simulink model "hrg_lift_tdm_shared"  (R2025a)
settings: Solver=FixedStepDiscrete  StartTime=0.0  StopTime=(floor(c.duration/L.T+1e-9)-1)*L.T  FixedStep=L.T  RelTol=1e-3
model workspace (MAT data in the model file):
  L.F = [0.999580432532 -1.0372095128e-09 6.81624270452e-05 6.2277917735e-05 1.75963318556e-117 1.36918786801e-121 -0.235732623336 -0.000170581053866 0.235732623336 0.000170581053866 8.59950268771e-05 -1.70759216614e-09 ... (676 elements, 26x26)]
  L.G = [-0.000674269741511 -4.08813584994e-07 0.00751103389356 -4.57676319434e-08 1.57194245886e-96 -1.68771046318e-124 -0.0205539124342 2.21019907253e-07 0.0205539124342 -2.21019907253e-07 -3.00124965015e-07 -2.89912617394e-11 ... (104 elements, 26x4)]
  L.Hm = [0.999684195246  -1.23947288142e-06  -4.2771939927e-05  -4.66937085047e-05  -1.75385746799e-05  -9.52623491396e-09  -2.77437214297e-15  -3.69811119948e-16  2.77437214289e-15  3.69811119948e-16  0  0  0  0  0  0  0  0  0  0  0  0  0  0  0  0; -1.23947288142e-06  0.999686910144  -4.66937085048e-05  5.9504357854e-05  -9.52623491397e-09  -1.75177087416e-05  -3.69811119948e-16  -1.96435054823e-15  3.69811119948e-16  1.96435054816e-15  0  0  0  0  0  0  0  0  0  0  0  0  0  0  0  0; 7.61670764012e-05  4.67132902328e-05  0.999689500075  3.71691546591e-06  0.000204402550454  -5.17736492516e-11  7.91753997903e-12  2.93241599996e-17  -7.91753997903e-12  -2.93241599996e-17  0  0  0  0  0  0  0  0  0  0  0  0  0  0  0  0; 4.67132902329e-05  -2.61521125254e-05  3.71691546591e-06  0.999681358669  -5.17736492516e-11  0.000204402663857  2.93241599996e-17  7.91747574839e-12  -2.93241599996e-17  -7.91747574839e-12  0  0  0  0  0  0  0  0  0  0  0  0  0  0  0  0]
  L.Jm = [-0.000674148886807  -2.90869128238e-07  -0.00751258628212  7.3251807826e-09; -2.90869128238e-07  -0.000673511777043  7.32518078263e-09  -0.00751260232694; 0.00751184791082  -7.35240363844e-09  -0.000674460705417  -2.94234049475e-07; -7.35240363847e-09  0.00751186401527  -2.94234049475e-07  -0.000673816225245]
  L.Hc = [0.999711481766  2.14384983506e-06  -6.12338918604e-05  -4.3067940708e-05  -1.75428280259e-05  -8.84421170948e-09  -2.92065727036e-15  -3.41103284536e-16  2.92065727027e-15  3.41103284536e-16  5.25450884933e-18  0  -5.25450884933e-18  0  3.30942182373e-19  0  -3.30942182373e-19  0  1.39036561883e-20  0  -1.39036561883e-20  0  2.92225038045e-22  0  -2.92225038045e-22  0; 2.14384983507e-06  0.99970678595  -4.3067940708e-05  3.31006484918e-05  -8.84421170949e-09  -1.75234559678e-05  -3.41103284536e-16  -2.17351633368e-15  3.41103284536e-16  2.17351633362e-15  0  5.25450884933e-18  0  -5.25450884933e-18  0  3.30942182373e-19  0  -3.30942182373e-19  0  1.39036561883e-20  0  -1.39036561883e-20  0  2.92225038045e-22  0  -2.92225038045e-22; 6.56554924056e-05  4.41462676728e-05  0.999704818384  2.39219219878e-06  0.000204405866873  -2.77622515808e-10  7.91766132564e-12  1.88386068823e-17  -7.91766132564e-12  -1.88386068823e-17  -8.14258443032e-18  0  8.14258443032e-18  0  -5.20771635647e-19  0  5.20771635647e-19  0  -2.22068360541e-20  0  2.22068360541e-20  0  -4.73526685999e-22  0  4.73526685999e-22  0; 4.41462676729e-05  -3.10409783354e-05  2.39219219878e-06  0.999699578606  -2.77622515808e-10  0.000204406474967  1.88386068823e-17  7.91762006219e-12  -1.88386068823e-17  -7.91762006219e-12  0  -8.14258443032e-18  0  8.14258443032e-18  0  -5.20771635647e-19  0  5.20771635647e-19  0  -2.22068360541e-20  0  2.22068360541e-20  0  -4.73526685999e-22  0  4.73526685999e-22]
  L.Jc = [-0.000674306006234  -2.65903485878e-07  -0.00751277889474  -2.05468037642e-08; -2.65903485878e-07  -0.000673723580356  -2.05468037642e-08  -0.00751273388972; 0.00751197010124  -1.55767638394e-08  -0.000674392037013  -2.74048667129e-07; -1.55767638394e-08  0.00751200422004  -2.74048667129e-07  -0.00067379177021]
  L.T = 0.000588235294118
  L.cvMap = [0 0 9.25181123354e-09 -1.72311612446e-14 1.45369811075e-07 -2.57068827924e-13 7.22706720145e-07 -1.21288024566e-12 2.24303510145e-06 -3.57018191525e-12 5.37764474432e-06 -8.11115525781e-12 ... (96000 elements, 3200x30)]
  L.candidateOffset_s = 0.000515625
  c.mode = 'tdm_shared'
  c.reuse = 1
  c.continuous = 0
  c.Ts = 1.83823529412e-07
  c.w = 42725.6600888
  c.omega = 0
  c.duration = 0.12
  c.B = 0.276990961962
  c.n = 800
  c.adcLatency = 5
  c.logDecimation = 1
  c.p.schema = 'v10.1'
  c.p.synthetic = 1
  c.p.f0 = 6800
  c.p.gamma_intrinsic = 0.712094334814
  c.p.Cs = 7.2e-10
  c.p.G0 = 1e-10
  c.p.kappa = 1e-06
  c.p.b = 1.1e-06
  c.p.Cds = 0
  c.p.Rs = 1000
  c.p.B = 0.276990961962
  c.p.Omega = 0
  c.p.Ts = 1.83823529412e-07
  c.p.Tc = 0.001
  c.p.duration = 0.12
  c.p.charge_target = 1e-11
  c.p.initial_fraction = 1
  c.p.theta0 = 0.785398163397
  c.p.Cf = 1e-10
  c.p.Rf = 1000000000
  c.p.driver_tau = [2e-06; 2e-06]
  c.p.afe_bw = [20000; 20000]
  c.p.detect_matrix = [1  0; 0  1]
  c.p.drive_matrix = [20  0; 0  20]
  c.p.split_hz = 0.05
  c.p.stiffness_axis = 0.37
  c.p.damping_half_difference = 0
  c.p.damping_axis = -0.23
  c.p.adc_span = 2
  c.p.adc_bits = 40
  c.p.dac_span = 1
  c.p.dac_bits = 40
  c.p.vmax = 0.5
  c.p.agc_bw = 10
  c.p.quad_bw = 4
  c.p.pll_gain = 30
  c.p.max_detune = 30
  c.p.virtual_rate = 0
  c.p.virtual_start_min_s = 0.25
  c.p.virtual_settle_fraction = 0.01
  c.p.predict_heading = 1
  c.p.max_heading_rate = 100
  c.p.virtual_validated_limit = 0.2
  c.p.min_amplitude_fraction = 0.02
  c.p.min_linearity = 0.1
  c.p.max_calibration_condition = 100
  c.p.max_frame_age = 0.002
  c.p.calibrate_detection = 1
  c.p.calibrate_drive = 1
  c.p.noise_rms_V = 0
  c.p.noise_seed = 52
  c.p.carrier_hz = 6800
  c.p.Q = 30000
  c.p.pre_gain = 1
  c.p.power_gain = 20
  c.p.aaf_order = 4
  c.p.fs = 5440000
  c.p.bleed_R = 2777.77854938
  c.p.reset_tau = 2e-06
  c.p.adc_latency = 5
  c.p.log_decimation = 200
  c.p.adc_noise_rms = 0
  c.p.adc_dither_lsb_rms = 0
  c.p.adc_dither_seeds = [1103515245; 2246822519]
  c.p.dac_divisor = 1
  c.p.allow_adc_underclock = 0
  c.p.seed_enabled = 0
  c.p.seed_seconds = 0.03
  c.p.seed_voltage = 0.2
  c.p.cv_mode = 'thx2024'
  c.p.thx_cv_gain = 10000
  c.p.thx_charge_per_input = 1e-06
  c.p.cv_source = 'thx2024'
  c.head.f0_Hz = 6800
  c.head.split_Hz = 0.05
  c.head.Q = 30000
  c.head.parasitic_F = 7.2e-10
  c.head.f_modes_Hz = [6799.975 6800.025]
  c.head.ringdown_s = 1.4043083214
  c.head.linewidth_Hz = 0.226666666667
  c.head.temperature_model = 'No per-head temperature curve supplied'
  c.head.group_shunt_F = [7.2e-10; 7.2e-10; 7.2e-10; 7.2e-10]
  c.driveEnd = 800
  c.senseStart = 1200
  c.validStart = 2000
  c.validEnd = 2800
  c.frame = 3200
  c.adcStep = 1.81898940355e-12
  c.adcMin = -1
  c.adcMax = 0.999999999998
  c.dacStep = 9.09494701773e-13
  c.dacMin = -0.5
  c.dacMax = 0.499999999999
  c.minEnergy = 0.0004
  c.minLinearity = 0.1
  c.agc = 62.8318530718
  c.gamma = 0.712094334814
  c.quad = 25.1327412287
  c.forceScale = 3.10732073373
  c.startCommand = [0; 0; 0; 0]
  c.seedCommand = [0; 0; -0.141421356237; -0.141421356237]
  c.stateCount = 26
  c.pickoff = [0  0  0  0  0  0  0  0  0  0  0  0  0  0  0  0  0  0  0  0  0  0  0.4  0  -0.4  0; 0  0  0  0  0  0  0  0  0  0  0  0  0  0  0  0  0  0  0  0  0  0  0  0.4  0  -0.4]
  c.motion = [1  0  0  0  0  0  0  0  0  0  0  0  0  0  0  0  0  0  0  0  0  0  0  0  0  0; 0  1  0  0  0  0  0  0  0  0  0  0  0  0  0  0  0  0  0  0  0  0  0  0  0  0]
  c.electrode = [0  0  0  0  0  0  0.000213628300444  0  -0.000213628300444  0  0  0  0  0  0  0  0  0  0  0  0  0  0  0  0  0; 0  0  0  0  0  0  0  0.000213628300444  0  -0.000213628300444  0  0  0  0  0  0  0  0  0  0  0  0  0  0  0  0]
  c.cvOutputGain = 10000
  c.Ad = [0.999969157815 1.52915577691e-10 -0.00785385721515 3.89392300717e-08 -4.8120754142e-24 1.18286541441e-29 7.54624297668e-05 -3.7414114096e-10 -7.54624297668e-05 3.7414114096e-10 0 0 ... (676 elements, 26x26)]
  c.Bd = [1.98586033351e-09  2.85360001372e-20; 2.85360001371e-20  1.98586033345e-09; 7.81249130157e-07  1.874197643e-17; 1.874197643e-17  7.81249130116e-07; 0.0878143670381  4.41008002219e-39; 2.74147144734e-39  0.0878143670381; 3956.34070317  -1.60514451093e-19; -1.60514451093e-19  3956.34070317; -3956.34070317  1.60514451093e-19; 1.60514451093e-19  -3956.34070317; 0  0; 0  0; 0  0; 0  0; 0  0; 0  0; 0  0; 0  0; 0  0; 0  0; 0  0; 0  0; 0  0; 0  0; 0  0; 0  0]
  c.Af = [0.999969157815 1.5291557769e-10 -0.00785385721504 3.89392300711e-08 0 0 0.000972567461954 -4.82198993752e-09 -0.000972567461954 4.82198993752e-09 0 0 ... (676 elements, 26x26)]
  c.As = [0.999969157815 1.5291557769e-10 -0.00785385721504 3.89392300711e-08 0 0 0.000922446324138 -4.57348880805e-09 -0.000922446324138 4.57348880805e-09 -0.0228351704558 -7.11424365435e-14 ... (676 elements, 26x26)]
  c.x0 = [0.707106781187; 0.707106781187; 0; 0; 0; 0; 0; 0; 0; 0; 0; 0; 0; 0; 0; 0; 0; 0; 0; 0; 0; 0; 0; 0; 0; 0]
  c.detect = [-0.353453438315  0  -1.51577588934  0; 0  -0.353453438315  0  -1.51577588934; 1.51577588934  0  -0.353453438315  0; 0  1.51577588934  0  -0.353453438315]
  c.drive = [0.0249907949795  0  0.00224213479427  0; 0  0.0249907949795  0  0.00224213479427; -0.00224213479427  0  0.0249907949795  0; 0  -0.00224213479427  0  0.0249907949795]
  c.gain_check.drive_pre_V_per_V = 1
  c.gain_check.sense_pre_V_per_V = 1
  c.gain_check.driver_post_gain = 20
  c.gain_check.detector_V_per_normalized_charge = 0.642491786495
  c.gain_check.electrode_limit_V = 10
  c.gain_check.drive_modal_V_per_command = 39.8546520136
  c.gain_check.drive_condition = 1
  c.gain_check.sense_condition = 1
  c.thx_comparison.saved_Kcvd = 10000
  c.thx_comparison.saved_Kcvs = 100000
  c.thx_comparison.saved_Kcsd = 10000
  c.thx_comparison.saved_Kcss = 100000
  c.thx_comparison.matched_cv_gain = 10000
  c.thx_comparison.piezo_charge_per_input_unit_C = 1e-06
  c.thx_comparison.reuse_scope = 'THX static readout Gain, matched to drive channel source value. Piezo adapter and AAF are external.'
  c.stateRows = {'1:4', '5:6', '7:10', '11:26'}
  c.portDriveMap = [1  0; 0  1; -1  0; 0  -1]
  c.portSenseMap = [4  0  -4  0; 0  4  0  -4]
  c.portCoupling = [1  0; 0  1; -1  0; 0  -1]
  c.portCapacitance_F = [7.2e-10  0  0  0; 0  7.2e-10  0  0; 0  0  7.2e-10  0; 0  0  0  7.2e-10]
  c.portShuntCapacitance_F = [7.2e-10; 7.2e-10; 7.2e-10; 7.2e-10]
  c.groupAngles_deg = [0; 45; 90; 135]
  c.groupNames = {'A', 'B', 'C', 'D'}
  c.commonTerminal = 'COM'
  c.portOptions.group_angles_deg = [0; 45; 90; 135]
  c.portOptions.group_charge_gain = [1; 1; 1; 1]
  c.portOptions.group_capacitance_F = [7.2e-10; 7.2e-10; 7.2e-10; 7.2e-10]
  c.portOptions.drive_on_resistance_ohm = 10
  c.portOptions.diagnostic_carrier_phase_rad = []
  c.portCV = [0  0  0  0  0  0  0  0  0  0  0  0  0  0  0  0  0  0  0  0  0  0  0.1  0  0  0; 0  0  0  0  0  0  0  0  0  0  0  0  0  0  0  0  0  0  0  0  0  0  0  0.1  0  0; 0  0  0  0  0  0  0  0  0  0  0  0  0  0  0  0  0  0  0  0  0  0  0  0  0.1  0; 0  0  0  0  0  0  0  0  0  0  0  0  0  0  0  0  0  0  0  0  0  0  0  0  0  0.1]
  c.groupVoltage = [0  0  0  0  0  0  0.000427256600888  0  0  0  0  0  0  0  0  0  0  0  0  0  0  0  0  0  0  0; 0  0  0  0  0  0  0  0.000427256600888  0  0  0  0  0  0  0  0  0  0  0  0  0  0  0  0  0  0; 0  0  0  0  0  0  0  0  0.000427256600888  0  0  0  0  0  0  0  0  0  0  0  0  0  0  0  0  0; 0  0  0  0  0  0  0  0  0  0.000427256600888  0  0  0  0  0  0  0  0  0  0  0  0  0  0  0  0]
  c.periodicCarrier = 1
settings Model: Creator=Administrator  LastModifiedBy=Administrator

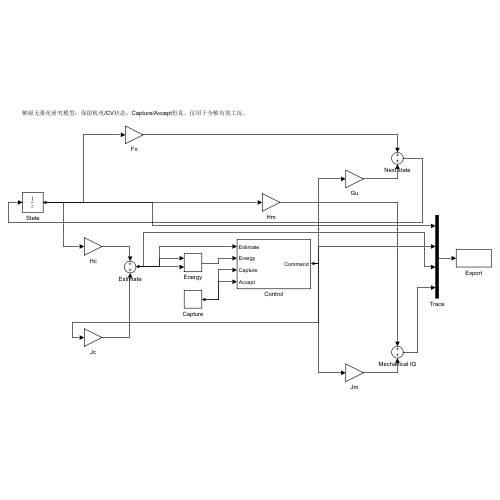
[thumbnail: Simulink's stored preview of the top-level diagram]
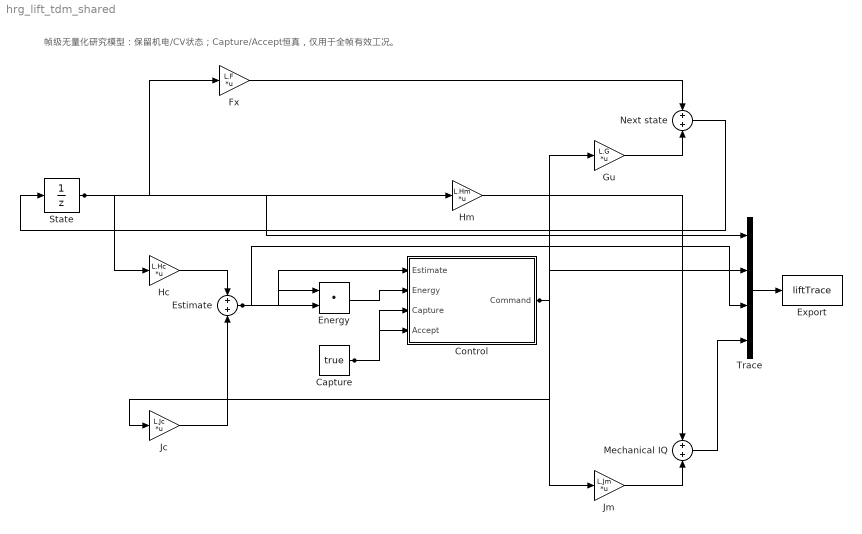
== system hrg_lift_tdm_shared ==
  note: 帧级无量化研究模型：保留机电/CV状态；Capture/Accept恒真，仅用于全帧有效工况。
  Capture : Constant  Value=true  OutDataTypeStr=boolean
  Control : Subsystem
  Energy : DotProduct  OutDataTypeStr=Inherit: Inherit via internal rule
  Estimate : Sum
  Export : ToWorkspace  VariableName=liftTrace  SampleTime=-1
  Fx : Gain  Gain=L.F  Multiplication=Matrix(K*u)
  Gu : Gain  Gain=L.G  Multiplication=Matrix(K*u)
  Hc : Gain  Gain=L.Hc  Multiplication=Matrix(K*u)
  Hm : Gain  Gain=L.Hm  Multiplication=Matrix(K*u)
  Jc : Gain  Gain=L.Jc  Multiplication=Matrix(K*u)
  Jm : Gain  Gain=L.Jm  Multiplication=Matrix(K*u)
  Mechanical IQ : Sum
  Next state : Sum
  State : UnitDelay  InitialCondition=c.x0  SampleTime=-1  HasFrameUpgradeWarning=on
  Trace : Mux
  wires:
  State/1 -> Fx/1, Hm/1, Trace/1, Hc/1
  Hm/1 -> Mechanical IQ/1
  Fx/1 -> Next state/1
  Hc/1 -> Estimate/1
  Estimate/1 -> Trace/3, Control/1(Estimate), Energy/1, Energy/2
  Jc/1 -> Estimate/2
  Energy/1 -> Control/2(Energy)
  Capture/1 -> Control/3(Capture), Control/4(Accept)
  Control/1(Command) -> Jc/1, Trace/2, Jm/1, Gu/1
  Gu/1 -> Next state/2
  Jm/1 -> Mechanical IQ/2
  Next state/1 -> State/1
  Mechanical IQ/1 -> Trace/4
  Trace/1 -> Export/1

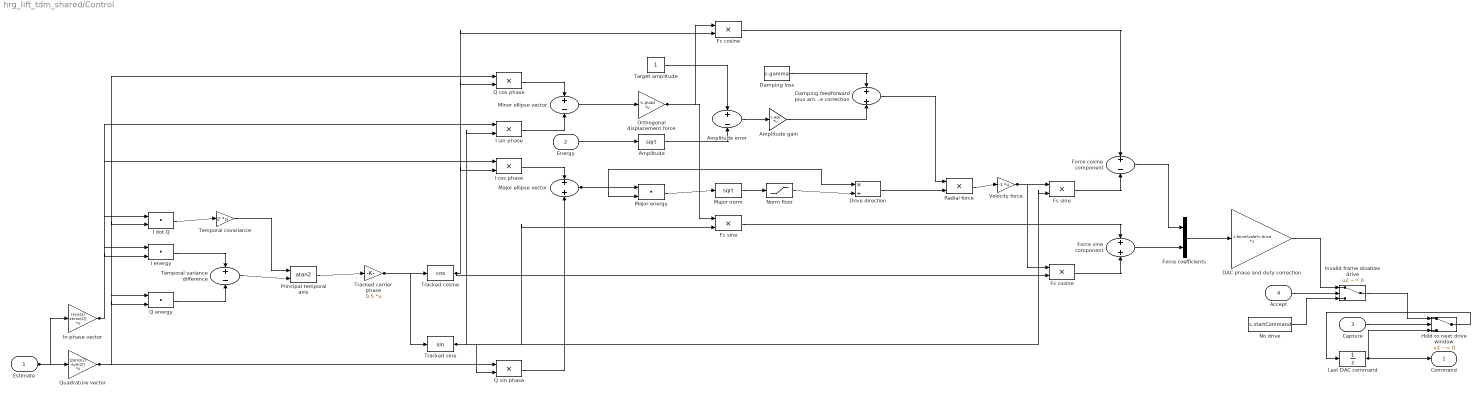
== system hrg_lift_tdm_shared/Control ==
  Estimate : Inport
  Energy : Inport  Port=2
  Capture : Inport  Port=3
  Accept : Inport  Port=4
  Amplitude : Sqrt
  Amplitude error : Sum  Inputs=+-
  Amplitude gain : Gain  Gain=c.agc  Multiplication=Matrix(K*u)
  DAC phase and duty correction : Gain  Gain=c.forceScale*c.drive  Multiplication=Matrix(K*u)
  Damping feedforward plus amplitude correction : Sum
  Damping loss : Constant  Value=c.gamma
  Drive direction : Product  Inputs=*/
  Fc cosine : Product
  Fc sine : Product
  Force coefficients : Mux  Inputs=2
  Force cosine component : Sum  Inputs=+-
  Force sine component : Sum
  Fs cosine : Product
  Fs sine : Product
  Hold to next drive window : Switch  Criteria=u2 ~= 0  SaturateOnIntegerOverflow=off  InputSameDT=off
  I cos phase : Product
  I dot Q : DotProduct  OutDataTypeStr=Inherit: Inherit via internal rule
  I energy : DotProduct  OutDataTypeStr=Inherit: Inherit via internal rule
  I sin phase : Product
  In-phase vector : Gain  Gain=[eye(2) zeros(2)]  Multiplication=Matrix(K*u)
  Invalid frame disables drive : Switch  Criteria=u2 ~= 0  SaturateOnIntegerOverflow=off  InputSameDT=off
  Last DAC command : UnitDelay  InitialCondition=c.startCommand  SampleTime=L.T  HasFrameUpgradeWarning=on
  Major ellipse vector : Sum
  Major energy : DotProduct  OutDataTypeStr=Inherit: Inherit via internal rule
  Major norm : Sqrt
  Minor ellipse vector : Sum  Inputs=+-
  No drive : Constant  Value=c.startCommand
  Norm floor : Saturate  UpperLimit=inf  LowerLimit=1e-9
  Orthogonal displacement force : Gain  Gain=-c.quad  Multiplication=Matrix(K*u)
  Principal temporal axis : Trigonometry  Operator=atan2
  Q cos phase : Product
  Q energy : DotProduct  OutDataTypeStr=Inherit: Inherit via internal rule
  Q sin phase : Product
  Quadrature vector : Gain  Gain=[zeros(2) eye(2)]  Multiplication=Matrix(K*u)
  Radial force : Product
  Target amplitude : Constant
  Temporal covariance : Gain  Gain=2  Multiplication=Matrix(K*u)
  Temporal variance difference : Sum  Inputs=+-
  Tracked carrier phase : Gain  Gain=0.5  Multiplication=Matrix(K*u)
  Tracked cosine : Trigonometry  Operator=cos
  Tracked sine : Trigonometry
  Velocity force : Gain  Gain=-1  Multiplication=Matrix(K*u)
  Command : Outport
  wires:
  Hold to next drive window/1 -> Last DAC command/1
  Last DAC command/1 -> Command/1, Hold to next drive window/3
  Invalid frame disables drive/1 -> Hold to next drive window/1
  Force sine component/1 -> Force coefficients/2
  Force cosine component/1 -> Force coefficients/1
  Fs sine/1 -> Force cosine component/2
  Velocity force/1 -> Fs cosine/1, Fs sine/1
  Radial force/1 -> Velocity force/1
  Drive direction/1 -> Radial force/2
  Damping feedforward plus amplitude correction/1 -> Radial force/1
  Damping loss/1 -> Damping feedforward plus amplitude correction/1
  Fc sine/1 -> Force sine component/1
  Amplitude error/1 -> Amplitude gain/1
  Fc cosine/1 -> Force cosine component/1
  Major energy/1 -> Major norm/1
  Amplitude/1 -> Amplitude error/2
  Orthogonal displacement force/1 -> Fc sine/1, Fc cosine/1
  Capture/1 -> Hold to next drive window/2
  Target amplitude/1 -> Amplitude error/1
  DAC phase and duty correction/1 -> Invalid frame disables drive/1
  Major ellipse vector/1 -> Major energy/1, Major energy/2, Drive direction/1
  Energy/1 -> Amplitude/1
  Minor ellipse vector/1 -> Orthogonal displacement force/1
  Amplitude gain/1 -> Damping feedforward plus amplitude correction/2
  Q sin phase/1 -> Major ellipse vector/2
  I sin phase/1 -> Minor ellipse vector/2
  Q cos phase/1 -> Minor ellipse vector/1
  I cos phase/1 -> Major ellipse vector/1
  Force coefficients/1 -> DAC phase and duty correction/1
  Tracked sine/1 -> I sin phase/2, Q sin phase/2, Fs sine/2, Fc sine/2
  Accept/1 -> Invalid frame disables drive/2
  Tracked cosine/1 -> Fs cosine/2, Q cos phase/2, I cos phase/2, Fc cosine/2
  Tracked carrier phase/1 -> Tracked cosine/1, Tracked sine/1
  Principal temporal axis/1 -> Tracked carrier phase/1
  Norm floor/1 -> Drive direction/2
  Q energy/1 -> Temporal variance difference/2
  I energy/1 -> Temporal variance difference/1
  I dot Q/1 -> Temporal covariance/1
  Temporal covariance/1 -> Principal temporal axis/1
  Quadrature vector/1 -> Q sin phase/1, Q cos phase/1, I dot Q/2, Q energy/2, Q energy/1
  Major norm/1 -> Norm floor/1
  Temporal variance difference/1 -> Principal temporal axis/2
  Estimate/1 -> Quadrature vector/1, In-phase vector/1
  Fs cosine/1 -> Force sine component/2
  No drive/1 -> Invalid frame disables drive/3
  In-phase vector/1 -> I cos phase/1, I energy/1, I dot Q/1, I energy/2, I sin phase/1
